simulink model "sf_change_detection_ramp"  (R2025b)
settings: Solver=FixedStepDiscrete  StartTime=0.0  StopTime=6  FixedStep=1  RelTol=1e-3  EnableMultiTasking=on
libraries: simulink x1
settings Model: Creator=The MathWorks, Inc.  LastModifiedBy=The MathWorks, Inc.
settings SolverCC: AlgebraicLoopSolver=TrustRegion
settings DataIOCC: LimitDataPoints=on  SaveFormat=Array  ReturnWorkspaceOutputs=off
settings OptimizationCC: ReuseModelBlockBuffer=off  ExpressionDepthLimit=2147483647.0  InitFltsAndDblsToZero=on  LifeSpan=inf
settings DebuggingCC: SaveWithParameterizedLinksMsg=none  UnderspecifiedInitializationDetection=Classic  MergeDetectMultiDrivingBlocksExec=none  SignalResolutionControl=TryResolveAllWithWarning  SolverPrmCheckMsg=warning  FcnCallInpInsideContextMsg=warning  UnconnectedInputMsg=warning  UnconnectedOutputMsg=warning  UnconnectedLineMsg=warning  StateNameClashWarn=warning  SFUnexpectedBacktrackingDiag=warning  SFNoUnconditionalDefaultTransitionDiag=warning  SFExecutionAtInitializationDiag=none  ArithmeticOperatorsInVariantConditions=warning
settings HardwareCC: ProdBitPerPointer=32.0  ProdBitPerSizeT=32.0  ProdBitPerPtrDiffT=32.0  ProdLargestAtomicFloat=None  ProdIntDivRoundTo=Undefined  ProdEndianess=Unspecified  ProdWordSize=32.0  ProdHWDeviceType=32-bit Generic
settings ModelReferenceCC: EnableRefExpFcnMdlSchedulingChecks=on  PropagateSignalLabelsOutOfModel=off
settings SFSimCC: SimUseLocalCustomCode=off  SimParseCustomCode=off  CustomCodeUndefinedFunction=UseInterfaceOnly
settings RTWCC: RTWUseLocalCustomCode=off  GPUComputeCapability=3.5
settings CodeAppCC: StateflowObjectComments=on
settings GRTTargetCC: TargetFcnLib=ansi_tfl_tmw.mat  TargetLangStandard=C89/C90 (ANSI)  CombineOutputUpdateFcns=off  GRTInterface=on
settings ConfigComp: CovMetricSettings=dw  CovSaveCumulativeToWorkspaceVar=on  CovSaveSingleToWorkspaceVar=on  CovExternalEMLEnable=off

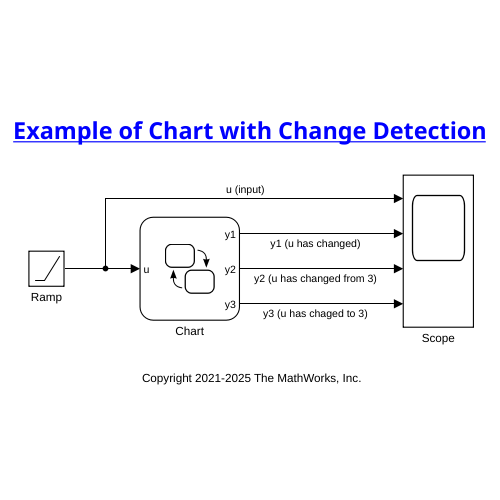
[thumbnail: Simulink's stored preview of the top-level diagram]
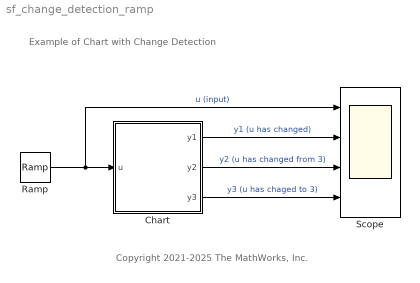
== system sf_change_detection_ramp ==
  note: Copyright 2021-2025 The MathWorks, Inc.
  note: Example of Chart with Change Detection
  Chart : Stateflow chart  TreatAsAtomicUnit=on
  Ramp : simulink/Sources/Ramp  slope=1  start=0  InitialOutput=0
  Scope : Scope  NumInputPorts=4
      settings: ActiveDisplayYMinimum=-0.625  ActiveDisplayYMaximum=5.625
  wires:
  Ramp/1 -> Scope/1, Chart/1(u)  "u (input)"
  Chart/1(y1) -> Scope/2  "y1 (u has changed)"
  Chart/2(y2) -> Scope/3  "y2 (u has changed from 3)"
  Chart/3(y3) -> Scope/4  "y3 (u has chaged to 3)"

== stateflow chart sf_change_detection_ramp/Chart ==
  (default) -> (junction 2) : {
      | y1 = hasChanged(u);
      | y2 = hasChangedFrom(u,3);
      | y3 = hasChangedTo(u,3);
      | }
  data: u input double; y1 output double; y2 output double; y3 output double
